simulink model "nms_sim_2D_cost"  (R2024b)
settings: Solver=ode15s  StartTime=0.0  StopTime=t_sim  MaxStep=dt_max  EnableMultiTasking=on
values from neighbouring files (symbols this model uses):
  a_BFSH = param_ctrl(35)*1    [setCtrlPar_optim_CPGreflex2001_2D.m]
  a_GAS = param_ctrl(37)*1    [setCtrlPar_optim_CPGreflex2001_2D.m]
  a_GLU = param_ctrl(31)*1    [setCtrlPar_optim_CPGreflex2001_2D.m]
  a_HAM = param_ctrl(33)*1    [setCtrlPar_optim_CPGreflex2001_2D.m]
  a_HFL = param_ctrl(32)*1    [setCtrlPar_optim_CPGreflex2001_2D.m]
  a_RF = param_ctrl(34)*1    [setCtrlPar_optim_CPGreflex2001_2D.m]
  a_SOL = param_ctrl(38)*1    [setCtrlPar_optim_CPGreflex2001_2D.m]
  a_TA = param_ctrl(39)*1    [setCtrlPar_optim_CPGreflex2001_2D.m]
  a_VAS = param_ctrl(36)*1    [setCtrlPar_optim_CPGreflex2001_2D.m]
  ai = param_ctrl(96)*2.0    [setCtrlPar_optim_CPGreflex2001_2D.m]
  b_BFSH = param_ctrl(52)*.51    [setCtrlPar_optim_CPGreflex2001_2D.m]
  b_BFSHGAS = param_ctrl(55)*.51    [setCtrlPar_optim_CPGreflex2001_2D.m]
  b_BFSHHAM = param_ctrl(54)*.51    [setCtrlPar_optim_CPGreflex2001_2D.m]
  b_BFSHVAS = param_ctrl(53)*.51    [setCtrlPar_optim_CPGreflex2001_2D.m]
  b_GAS = param_ctrl(59)*.51    [setCtrlPar_optim_CPGreflex2001_2D.m]
  b_GASBFSH = param_ctrl(60)*.51    [setCtrlPar_optim_CPGreflex2001_2D.m]
  b_GASSOL = param_ctrl(61)*.51    [setCtrlPar_optim_CPGreflex2001_2D.m]
  b_GLU = param_ctrl(40)*.51    [setCtrlPar_optim_CPGreflex2001_2D.m]
  b_GLUHAM = param_ctrl(42)*.51    [setCtrlPar_optim_CPGreflex2001_2D.m]
  b_GLUHFL = param_ctrl(41)*.51    [setCtrlPar_optim_CPGreflex2001_2D.m]
  b_HAM = param_ctrl(46)*.51    [setCtrlPar_optim_CPGreflex2001_2D.m]
  b_HAMBFSH = param_ctrl(48)*.51    [setCtrlPar_optim_CPGreflex2001_2D.m]
  b_HAMGLU = param_ctrl(47)*.51    [setCtrlPar_optim_CPGreflex2001_2D.m]
  b_HFL = param_ctrl(43)*.51    [setCtrlPar_optim_CPGreflex2001_2D.m]
  b_HFLGLU = param_ctrl(44)*.51    [setCtrlPar_optim_CPGreflex2001_2D.m]
  b_HFLRF = param_ctrl(45)*.51    [setCtrlPar_optim_CPGreflex2001_2D.m]
  b_RF = param_ctrl(49)*.51    [setCtrlPar_optim_CPGreflex2001_2D.m]
  b_RFHFL = param_ctrl(50)*.51    [setCtrlPar_optim_CPGreflex2001_2D.m]
  b_RFVAS = param_ctrl(51)*.51    [setCtrlPar_optim_CPGreflex2001_2D.m]
  b_SOL = param_ctrl(62)*.51    [setCtrlPar_optim_CPGreflex2001_2D.m]
  b_SOLGAS = param_ctrl(64)*.51    [setCtrlPar_optim_CPGreflex2001_2D.m]
  b_SOLTA = param_ctrl(63)*.51    [setCtrlPar_optim_CPGreflex2001_2D.m]
  b_TA = param_ctrl(65)*.51    [setCtrlPar_optim_CPGreflex2001_2D.m]
  b_TASOL = param_ctrl(66)*.51    [setCtrlPar_optim_CPGreflex2001_2D.m]
  b_VAS = param_ctrl(56)*.51    [setCtrlPar_optim_CPGreflex2001_2D.m]
  b_VASBFSH = param_ctrl(57)*.51    [setCtrlPar_optim_CPGreflex2001_2D.m]
  b_VASRF = param_ctrl(58)*.51    [setCtrlPar_optim_CPGreflex2001_2D.m]
  bias = param_ctrl(97)*2.5    [setCtrlPar_optim_CPGreflex2001_2D.m]
  c = 0.05    [nms_MS_2D_scaled.m]
  c_jointstop = 0.3 / (pi/180)    (= 17.1887338539)    [nms_MS_2D_scaled.m]
  D12_F = 0.16    *scaleL_JPhys    [nms_MechInit_2D_scaleSkel.m]
  D12_S = 0.2460	*sub_height    [nms_MechInit_2D_scaleSkel.m]
  D12_T = 0.2450  *sub_height    [nms_MechInit_2D_scaleSkel.m]
  D12y_F = 0.039  *sub_height    [nms_MechInit_2D_scaleSkel.m]
  D12z_HAT = 0.1    [nms_MS_2D_scaled.m]
  D13_F = 0.20    *scaleL_JPhys    [nms_MechInit_2D_scaleSkel.m]
  D1G_F = 0.14    *scaleL_JPhys    [nms_MechInit_2D_scaleSkel.m]
  D1G_HAT = 0.35  *scaleL_JPhys    [nms_MechInit_2D_scaleSkel.m]
  D1G_S = (0.3 - D12y_F/4)	*scaleL_JPhys    [nms_MechInit_2D_scaleSkel.m]
  D1G_T = (0.3 - D12y_F/4)	*scaleL_JPhys    [nms_MechInit_2D_scaleSkel.m]
  D1Gy_F = D12y_F*D1G_F/D12_F    (= 0.07)    [nms_MechInit_2D_scaleSkel.m]
  d_BFSH = param_ctrl(26)*1    [setCtrlPar_optim_CPGreflex2001_2D.m]
  d_GAS = param_ctrl(28)*1    [setCtrlPar_optim_CPGreflex2001_2D.m]
  d_GLU = param_ctrl(22)*1    [setCtrlPar_optim_CPGreflex2001_2D.m]
  d_HAM = param_ctrl(24)*1    [setCtrlPar_optim_CPGreflex2001_2D.m]
  d_HFL = param_ctrl(23)*1    [setCtrlPar_optim_CPGreflex2001_2D.m]
  d_RF = param_ctrl(25)*1    [setCtrlPar_optim_CPGreflex2001_2D.m]
  d_SOL = param_ctrl(29)*1    [setCtrlPar_optim_CPGreflex2001_2D.m]
  d_TA = param_ctrl(30)*1    [setCtrlPar_optim_CPGreflex2001_2D.m]
  d_VAS = param_ctrl(27)*1    [setCtrlPar_optim_CPGreflex2001_2D.m]
  DeltaThRef = 5e-3    (= 0.005)    [nms_MS_2D_scaled.m]
  dloptBFSH = 3.0    (= 3)    [setCtrlPar_optim_CPGreflex2001_2D.m]
  dloptGAS = 3.0    (= 3)    [setCtrlPar_optim_CPGreflex2001_2D.m]
  dloptGLU = 3.0    (= 3)    [setCtrlPar_optim_CPGreflex2001_2D.m]
  dloptHAM = 3.0    (= 3)    [setCtrlPar_optim_CPGreflex2001_2D.m]
  dloptHFL = 3.0    (= 3)    [setCtrlPar_optim_CPGreflex2001_2D.m]
  dloptRF = 3.0    (= 3)    [setCtrlPar_optim_CPGreflex2001_2D.m]
  dloptSOL = 3.0    (= 3)    [setCtrlPar_optim_CPGreflex2001_2D.m]
  dloptTA = 3.0    (= 3)    [setCtrlPar_optim_CPGreflex2001_2D.m]
  dloptVAS = 3.0    (= 3)    [setCtrlPar_optim_CPGreflex2001_2D.m]
  ec_BFSH = param_ctrl(80)*0.15    [setCtrlPar_optim_CPGreflex2001_2D.m]
  ec_GAS = param_ctrl(82)*0.15    [setCtrlPar_optim_CPGreflex2001_2D.m]
  ec_GLU = param_ctrl(76)*0.15    [setCtrlPar_optim_CPGreflex2001_2D.m]
  ec_HAM = param_ctrl(78)*0.15    [setCtrlPar_optim_CPGreflex2001_2D.m]
  ec_HFL = param_ctrl(77)*0.15    [setCtrlPar_optim_CPGreflex2001_2D.m]
  ec_RF = param_ctrl(79)*0.15    [setCtrlPar_optim_CPGreflex2001_2D.m]
  ec_TA = param_ctrl(84)*0.15    [setCtrlPar_optim_CPGreflex2001_2D.m]
  ec_VAS = param_ctrl(81)*0.15    [setCtrlPar_optim_CPGreflex2001_2D.m]
  eref = 0.04    [nms_MS_2D_scaled.m]
  eref_GAS = 0.1    [nms_MS_2D_scaled.m]
  eref_SOL = 0.1    [nms_MS_2D_scaled.m]
  es_BFSH = param_ctrl(89)*0.15    [setCtrlPar_optim_CPGreflex2001_2D.m]
  es_GAS = param_ctrl(91)*0.15    [setCtrlPar_optim_CPGreflex2001_2D.m]
  es_GLU = param_ctrl(85)*0.15    [setCtrlPar_optim_CPGreflex2001_2D.m]
  es_HAM = param_ctrl(87)*0.15    [setCtrlPar_optim_CPGreflex2001_2D.m]
  es_HFL = param_ctrl(86)*0.15    [setCtrlPar_optim_CPGreflex2001_2D.m]
  es_RF = param_ctrl(88)*0.15    [setCtrlPar_optim_CPGreflex2001_2D.m]
  es_TA = param_ctrl(93)*0.15    [setCtrlPar_optim_CPGreflex2001_2D.m]
  es_VAS = param_ctrl(90)*0.15    [setCtrlPar_optim_CPGreflex2001_2D.m]
  FmaxBFSH = 350    [nms_MS_2D_scaled.m]
  FmaxGAS = 2000    [nms_MS_2D_scaled.m]
  FmaxGLU = 4000    [nms_MS_2D_scaled.m]
  FmaxHAM = 2000    [nms_MS_2D_scaled.m]
  FmaxHFL = 2000    [nms_MS_2D_scaled.m]
  FmaxRF = 850    [nms_MS_2D_scaled.m]
  FmaxSOL = 4000    [nms_MS_2D_scaled.m]
  FmaxTA = 800    [nms_MS_2D_scaled.m]
  FmaxVAS = 5000    [nms_MS_2D_scaled.m]
  g = 9.81    [nms_MS_2D_scaled.m]
  gamma_4 = param_ctrl(11) * 1.7    [setCtrlPar_optim_CPGreflexsynergy2023_2D.m]
  h_BFSH = param_ctrl(71)*.1    [setCtrlPar_optim_CPGreflex2001_2D.m]
  h_GAS = param_ctrl(73)*.1    [setCtrlPar_optim_CPGreflex2001_2D.m]
  h_GLU = param_ctrl(67)*.1    [setCtrlPar_optim_CPGreflex2001_2D.m]
  h_HAM = param_ctrl(69)*.1    [setCtrlPar_optim_CPGreflex2001_2D.m]
  h_HFL = param_ctrl(68)*.1    [setCtrlPar_optim_CPGreflex2001_2D.m]
  h_RF = param_ctrl(70)*.1    [setCtrlPar_optim_CPGreflex2001_2D.m]
  h_SOL = param_ctrl(74)*.1    [setCtrlPar_optim_CPGreflex2001_2D.m]
  h_TA = param_ctrl(75)*.1    [setCtrlPar_optim_CPGreflex2001_2D.m]
  h_VAS = param_ctrl(72)*.1    [setCtrlPar_optim_CPGreflex2001_2D.m]
  HLCtrlPar = [theta_tgt l_clr alpha_tgt alpha_cd alpha_cv]    [setCtrlPar_optim_reflex2015_2D.m]
  In_F = 0.005    *scaleM*scaleL_JPhys^2    [nms_MechInit_2D_scaleSkel.m]
  In_HAT = 2.5    *scaleM*scaleL_JPhys^2    [nms_MechInit_2D_scaleSkel.m]
  In_S = 0.05     *scaleM*scaleL_JPhys^2    [nms_MechInit_2D_scaleSkel.m]
  In_T = 0.15     *scaleM*scaleL_JPhys^2    [nms_MechInit_2D_scaleSkel.m]
  init_exc = 0.01    [setInitPar_optim_2D.m]
  init_fm = 0.01    [setInitPar_optim_2D.m]
  init_lce = 1    [setInitPar_optim_2D.m]
  init_LCPG = param_ctrl(12) * 0.01    [setCtrlPar_optim_CPGreflexsynergy2023_2D.m]
  init_LStance = 1    [setInitPar_optim_2D.m]
  init_N1 = osc_signal1(phi_off_osc_ind)    [setCtrlPar_optim_CPGreflex2001_2D.m]
  ... (+441 more)
undefined symbols (not defined in the file or in its folder): cost_act_exponent, cost_v_tgt, flag_controller, Newton, nStep_obj, nStep_startKin, Raphson, sgn, SSW_kin, terrain_slope_angle, v_plateS1, X, Y, Z
libraries: nesl_utility x94, sm_lib x90, simulink x28, simulink_extras x12
(part 20 of 20)

== system nms_sim_2D_cost/Body Mechanics/RHeel Contact/2D Contact/Static Friction Model ==
  note: Stiction Limit Detector
  note: Static Friction Model
  note: Zero multiplication prevents
      | horizontal friction model from
      | oscillating between static and kinetic
      | friction when the vertical force is zero but
      | the ground level is not yet reached
      | in the upward motion
  note: (distance to
      | surface)
  note: Tangential Ground Reaction Force
  pos [m] : Inport
  vel [m/s m/s] : Inport  Port=2
  RefPtFP [m m] : Inport  Port=3
  posFP [m] : Inport  Port=4
  nVecFP [m m] : Inport  Port=5
  Enable : EnablePort  StatesWhenEnabling=reset  ZeroCross=off
  Abs : Abs  SaturateOnIntegerOverflow=off
  Check Vertical Friction : Product  RndMeth=Zero
  Constant : Constant
  Dpos_n : DotProduct  OutDataTypeStr=Inherit: Inherit via internal rule
  Dpos_nVec : Product  RndMeth=Zero
  Dpos_tVec : Sum  Inputs=|+-
  FixPt Relational Operator : RelationalOperator  Operator=>  OutDataTypeStr=boolean  ZeroCross=off  InputSameDT=off
  Gain : Gain  Gain=-1
  Gain1 : Gain  Gain=k_gn
  Gain2 : Gain  Gain=1/v_gn_max
  Gain3 : Gain  Gain=k_gt
  Gain5 : Gain  Gain=1/v_gt_max
  Memory : Memory
  Mux2 : Mux  Inputs=2
  Normal Ground Reaction Force : Fcn  Expr="u(1)  *  (1-u(2)) * (u(2)<1)"
  Positive : simulink/Logic and Bit Operations/Compare To Zero  relop=>  OutDataTypeStr=boolean
  Positive1 : simulink/Logic and Bit Operations/Compare To Zero  relop=>  OutDataTypeStr=boolean
  Product1 : Product  RndMeth=Zero
  Sign : Signum  ZeroCross=off
  Sum : Sum  Inputs=-+
  Sum1 : Sum  Inputs=|+-
  Sum2 : Sum  Inputs=|+-
  Vector Norm : Subsystem
  d_n : DotProduct  OutDataTypeStr=Inherit: Inherit via internal rule
  stiction limit force : Gain  Gain=mu_stick
  sum : Sum  Inputs=++|
  tVec1 : Product  Inputs=**  RndMeth=Zero
  tVec2 : Product  Inputs=**  RndMeth=Zero
  v_n : DotProduct  OutDataTypeStr=Inherit: Inherit via internal rule
  v_nVec : Product  RndMeth=Zero
  v_tVec : Sum  Inputs=-+|
  F_n Stick [N N] : Outport  OutputWhenDisabled=reset  InitialOutput=[0 0]  VectorParamsAs1DForOutWhenUnconnected=off
      settings: AttributesFormatString=initial = '%<InitialOutput>'\nwhen disabled = '%<OutputWhenDisabled>'
  F_t Stick [N N] : Outport  Port=2  OutputWhenDisabled=reset  InitialOutput=[0 0]  VectorParamsAs1DForOutWhenUnconnected=off
      settings: AttributesFormatString=when disabled: %<OutputWhenDisabled>\ninitial: %<InitialOutput>
  Sliding! : Outport  Port=3  OutputWhenDisabled=reset  InitialOutput=0  VectorParamsAs1DForOutWhenUnconnected=off
      settings: AttributesFormatString=when disabled: %<OutputWhenDisabled>\ninitial: %<InitialOutput>
  wires:
  Sum/1 -> Positive/1
  Memory/1 -> FixPt Relational Operator/2
  Positive/1 -> FixPt Relational Operator/1, Memory/1
  FixPt Relational Operator/1 -> Sliding!/1
  Abs/1 -> Sum/1
  stiction limit force/1 -> Abs/1
  Positive1/1 -> Check Vertical Friction/2
  Check Vertical Friction/1 -> Vector Norm/1(vec), F_t Stick [N N]/1
  Normal Ground Reaction Force/1 -> Product1/2, stiction limit force/1, Positive1/1
  Mux2/1 -> Normal Ground Reaction Force/1
  Gain1/1 -> Mux2/1
  Gain2/1 -> Mux2/2
  nVecFP [m m]/1 -> d_n/1, v_n/2, Dpos_n/1, Dpos_nVec/1, v_nVec/2, Product1/1
  d_n/1 -> Gain1/1
  vel [m/s m/s]/1 -> v_tVec/2, v_n/1
  v_n/1 -> v_nVec/1, Gain2/1
  v_nVec/1 -> v_tVec/1
  v_tVec/1 -> Gain5/1
  Product1/1 -> F_n Stick [N N]/1
  pos [m]/1 -> Sum2/1, Sum1/2
  posFP [m]/1 -> Sum2/2
  Sum2/1 -> Dpos_n/2, Dpos_tVec/1  "Dpos"
  Dpos_n/1 -> Dpos_nVec/2
  Dpos_nVec/1 -> Dpos_tVec/2
  Dpos_tVec/1 -> Gain3/1
  Gain3/1 -> Sign/1, tVec2/2
  Sign/1 -> tVec1/2
  tVec1/1 -> sum/2
  Constant/1 -> sum/1
  sum/1 -> tVec2/1
  tVec2/1 -> Gain/1
  Gain/1 -> Check Vertical Friction/1
  Vector Norm/1(norm) -> Sum/2
  RefPtFP [m m]/1 -> Sum1/1
  Sum1/1 -> d_n/2
  Gain5/1 -> tVec1/1

== system nms_sim_2D_cost/CPG-reflex-synergy controller/Central Pattern Generator/Left Central Pattern Generator/Pulse 0 ==
  phi out : Inport
  Constant : Constant  Value=u1
  Constant1 : Constant
  Cos : Trigonometry  Operator=cos
  Gain : Gain  Gain=pi/sigma1
  Gain1 : Gain  Gain=0.5
  Scope{,1..3} (4 alike) : Scope
  Sum : Sum  Inputs=|+-
  Sum1 : Sum  Inputs=|++
  Out1 : Outport
  wires:
  phi out/1 -> Sum/1
  Constant/1 -> Sum/2
  Sum/1 -> Scope/1, Gain/1
  Gain/1 -> Scope1/1, Cos/1
  Constant1/1 -> Sum1/2
  Cos/1 -> Scope2/1, Sum1/1
  Sum1/1 -> Scope3/1, Gain1/1
  Gain1/1 -> Out1/1

== system nms_sim_2D_cost/CPG-reflex-synergy controller/Central Pattern Generator/Left Central Pattern Generator/Pulse 1 ==
  phi out : Inport
  Constant : Constant  Value=u2
  Constant1 : Constant
  Cos : Trigonometry  Operator=cos
  Gain : Gain  Gain=pi/sigma2
  Gain1 : Gain  Gain=0.5
  Scope{,1..3} (4 alike) : Scope
  Sum : Sum  Inputs=|+-
  Sum1 : Sum  Inputs=|++
  Out1 : Outport
  wires:
  Gain1/1 -> Out1/1
  Sum1/1 -> Gain1/1, Scope3/1
  Cos/1 -> Sum1/1, Scope2/1
  Constant1/1 -> Sum1/2
  Gain/1 -> Cos/1, Scope1/1
  Sum/1 -> Gain/1, Scope/1
  Constant/1 -> Sum/2
  phi out/1 -> Sum/1

== system nms_sim_2D_cost/CPG-reflex-synergy controller/Central Pattern Generator/Left Central Pattern Generator/Pulse 2 ==
  phi out : Inport
  Constant : Constant  Value=u3
  Constant1 : Constant
  Cos : Trigonometry  Operator=cos
  Gain : Gain  Gain=pi/sigma3
  Gain1 : Gain  Gain=0.5
  Scope{,1..3} (4 alike) : Scope
  Sum : Sum  Inputs=|+-
  Sum1 : Sum  Inputs=|++
  Out1 : Outport
  wires:
  phi out/1 -> Sum/1
  Constant/1 -> Sum/2
  Sum/1 -> Scope/1, Gain/1
  Gain/1 -> Scope1/1, Cos/1
  Constant1/1 -> Sum1/2
  Cos/1 -> Scope2/1, Sum1/1
  Sum1/1 -> Scope3/1, Gain1/1
  Gain1/1 -> Out1/1

== system nms_sim_2D_cost/CPG-reflex-synergy controller/Central Pattern Generator/Left Central Pattern Generator/Pulse 3 ==
  phi out : Inport
  Constant : Constant  Value=u4
  Constant1 : Constant
  Cos : Trigonometry  Operator=cos
  Gain : Gain  Gain=pi/sigma4
  Gain1 : Gain  Gain=0.5
  Scope{,1..3} (4 alike) : Scope
  Sum : Sum  Inputs=|+-
  Sum1 : Sum  Inputs=|++
  Out1 : Outport
  wires:
  Gain1/1 -> Out1/1
  Sum1/1 -> Gain1/1, Scope3/1
  Cos/1 -> Sum1/1, Scope2/1
  Constant1/1 -> Sum1/2
  Gain/1 -> Cos/1, Scope1/1
  Sum/1 -> Gain/1, Scope/1
  Constant/1 -> Sum/2
  phi out/1 -> Sum/1

== system nms_sim_2D_cost/CPG-reflex-synergy controller/Central Pattern Generator/Left Central Pattern Generator/Pulse 4 ==
  phi out : Inport
  Constant : Constant  Value=u5
  Constant1 : Constant
  Cos : Trigonometry  Operator=cos
  Gain : Gain  Gain=pi/sigma5
  Gain1 : Gain  Gain=0.5
  Scope{,1..3} (4 alike) : Scope
  Sum : Sum  Inputs=|+-
  Sum1 : Sum  Inputs=|++
  Out1 : Outport
  wires:
  phi out/1 -> Sum/1
  Constant/1 -> Sum/2
  Sum/1 -> Scope/1, Gain/1
  Gain/1 -> Scope1/1, Cos/1
  Constant1/1 -> Sum1/2
  Cos/1 -> Scope2/1, Sum1/1
  Sum1/1 -> Scope3/1, Gain1/1
  Gain1/1 -> Out1/1

== system nms_sim_2D_cost/CPG-reflex-synergy controller/Central Pattern Generator/Right Central Pattern Generator/Pulse 0 ==
  phi out : Inport
  Constant : Constant  Value=u1
  Constant1 : Constant
  Cos : Trigonometry  Operator=cos
  Gain : Gain  Gain=pi/sigma1
  Gain1 : Gain  Gain=0.5
  Scope{,1..3} (4 alike) : Scope
  Sum : Sum  Inputs=|+-
  Sum1 : Sum  Inputs=|++
  Out1 : Outport
  wires:
  Gain1/1 -> Out1/1
  Sum1/1 -> Gain1/1, Scope3/1
  Cos/1 -> Sum1/1, Scope2/1
  Constant1/1 -> Sum1/2
  Gain/1 -> Cos/1, Scope1/1
  Sum/1 -> Gain/1, Scope/1
  Constant/1 -> Sum/2
  phi out/1 -> Sum/1

== system nms_sim_2D_cost/CPG-reflex-synergy controller/Central Pattern Generator/Right Central Pattern Generator/Pulse 1 ==
  phi out : Inport
  Constant : Constant  Value=u2
  Constant1 : Constant
  Cos : Trigonometry  Operator=cos
  Gain : Gain  Gain=pi/sigma2
  Gain1 : Gain  Gain=0.5
  Scope{,1..3} (4 alike) : Scope
  Sum : Sum  Inputs=|+-
  Sum1 : Sum  Inputs=|++
  Out1 : Outport
  wires:
  phi out/1 -> Sum/1
  Constant/1 -> Sum/2
  Sum/1 -> Scope/1, Gain/1
  Gain/1 -> Scope1/1, Cos/1
  Constant1/1 -> Sum1/2
  Cos/1 -> Scope2/1, Sum1/1
  Sum1/1 -> Scope3/1, Gain1/1
  Gain1/1 -> Out1/1

== system nms_sim_2D_cost/CPG-reflex-synergy controller/Central Pattern Generator/Right Central Pattern Generator/Pulse 2 ==
  phi out : Inport
  Constant : Constant  Value=u3
  Constant1 : Constant
  Cos : Trigonometry  Operator=cos
  Gain : Gain  Gain=pi/sigma3
  Gain1 : Gain  Gain=0.5
  Scope{,1..3} (4 alike) : Scope
  Sum : Sum  Inputs=|+-
  Sum1 : Sum  Inputs=|++
  Out1 : Outport
  wires:
  Gain1/1 -> Out1/1
  Sum1/1 -> Gain1/1, Scope3/1
  Cos/1 -> Sum1/1, Scope2/1
  Constant1/1 -> Sum1/2
  Gain/1 -> Cos/1, Scope1/1
  Sum/1 -> Gain/1, Scope/1
  Constant/1 -> Sum/2
  phi out/1 -> Sum/1

== system nms_sim_2D_cost/CPG-reflex-synergy controller/Central Pattern Generator/Right Central Pattern Generator/Pulse 3 ==
  phi out : Inport
  Constant : Constant  Value=u4
  Constant1 : Constant
  Cos : Trigonometry  Operator=cos
  Gain : Gain  Gain=pi/sigma4
  Gain1 : Gain  Gain=0.5
  Scope{,1..3} (4 alike) : Scope
  Sum : Sum  Inputs=|+-
  Sum1 : Sum  Inputs=|++
  Out1 : Outport
  wires:
  phi out/1 -> Sum/1
  Constant/1 -> Sum/2
  Sum/1 -> Scope/1, Gain/1
  Gain/1 -> Scope1/1, Cos/1
  Constant1/1 -> Sum1/2
  Cos/1 -> Scope2/1, Sum1/1
  Sum1/1 -> Scope3/1, Gain1/1
  Gain1/1 -> Out1/1

== system nms_sim_2D_cost/CPG-reflex-synergy controller/Central Pattern Generator/Right Central Pattern Generator/Pulse 4 ==
  phi out : Inport
  Constant : Constant  Value=u5
  Constant1 : Constant
  Cos : Trigonometry  Operator=cos
  Gain : Gain  Gain=pi/sigma5
  Gain1 : Gain  Gain=0.5
  Scope{,1..3} (4 alike) : Scope
  Sum : Sum  Inputs=|+-
  Sum1 : Sum  Inputs=|++
  Out1 : Outport
  wires:
  Gain1/1 -> Out1/1
  Sum1/1 -> Gain1/1, Scope3/1
  Cos/1 -> Sum1/1, Scope2/1
  Constant1/1 -> Sum1/2
  Gain/1 -> Cos/1, Scope1/1
  Sum/1 -> Gain/1, Scope/1
  Constant/1 -> Sum/2
  phi out/1 -> Sum/1

== system nms_sim_2D_cost/Reflex Controller/Lower Control Layer (Spinal Cord)/L Swing Phase/kneei_flexion from alpha ==
  note: Knee Phase i
  SBFSH : Inport
  Enable : EnablePort  StatesWhenEnabling=reset  ZeroCross=off
  SBFSH_Sw_ki : Outport  OutputWhenDisabled=reset  InitialOutput=0  VectorParamsAs1DForOutWhenUnconnected=off
  wires:
  SBFSH/1 -> SBFSH_Sw_ki/1

== system nms_sim_2D_cost/Reflex Controller/Lower Control Layer (Spinal Cord)/L Swing Phase/kneeii_damp and hold & kneeiii_leg stop & kneeiv_stance preparation ==
  note: Knee Phase i
  CtrlPar : Inport
  a_tgt : Inport  Port=2
  LceRF : Inport  Port=3
  LceHAM : Inport  Port=4
  VceHAM : Inport  Port=5
  VceVAS : Inport  Port=6
  VceBFSH : Inport  Port=7
  VceRF : Inport  Port=8
  LceHFL : Inport  Port=9
  LceGLU : Inport  Port=10
  LceVAS : Inport  Port=11
  Enable : EnablePort  StatesWhenEnabling=reset  ZeroCross=off
  Compare To Constant : simulink/Logic and Bit Operations/Compare To Constant  relop=<=  const=0  OutDataTypeStr=uint8  ZeroCross=off
  Constant1 : Constant  Value=0  OutDataTypeStr=boolean
  Constant2 : Constant  Value=0  OutDataTypeStr=boolean
  Constant3 : Constant  Value=0  OutDataTypeStr=boolean
  Constant4 : Constant
  Constant5 : Constant
  Demux1 : Demux  Outputs=5
  Divide1 : Product
  Divide2 : Product
  Logical Operator : Logic  Operator=NOT  AllPortsSameDT=off  OutDataTypeStr=boolean
  Logical Operator1 : Logic  AllPortsSameDT=off  OutDataTypeStr=boolean
  Relational Operator : RelationalOperator  Operator=<=  OutDataTypeStr=boolean  ZeroCross=off  InputSameDT=off
  Relational Operator1 : RelationalOperator  OutDataTypeStr=boolean  ZeroCross=off  InputSameDT=off
  S-R Flip-Flop : simulink_extras/Flip Flops/S-R Flip-Flop  initial_condition=0
  S-R Flip-Flop1 : simulink_extras/Flip Flops/S-R Flip-Flop  initial_condition=0
  S-R Flip-Flop2 : simulink_extras/Flip Flops/S-R Flip-Flop  initial_condition=0
  Sum1 : Sum  Inputs=+-|  InputSameDT=on  SaturateOnIntegerOverflow=on  OutDataTypeStr=Inherit: Same as first input
  Sum2 : Sum  Inputs=++|  InputSameDT=on  SaturateOnIntegerOverflow=on  OutDataTypeStr=Inherit: Same as first input
  Sum3 : Sum  Inputs=+-|  InputSameDT=on  SaturateOnIntegerOverflow=on  OutDataTypeStr=Inherit: Same as first input
  Sum4 : Sum  Inputs=+-|  InputSameDT=on  SaturateOnIntegerOverflow=on  OutDataTypeStr=Inherit: Same as first input
  Sum5 : Sum  Inputs=++|  InputSameDT=on  SaturateOnIntegerOverflow=on  OutDataTypeStr=Inherit: Same as first input
  Terminator : Terminator
  Terminator1 : Terminator
  Terminator2 : Terminator
  kneeii_damp and hold : Subsystem  TreatAsAtomicUnit=on
  kneeiii_leg stop : Subsystem  TreatAsAtomicUnit=on
  kneeiv_stance preparation : Subsystem  TreatAsAtomicUnit=on
  parSwKii : Selector  InputPortWidth=Sw_i  IndexOptions=Index vector (dialog)  Indices=parSwKii_i  OutputSizes=1
  parSwKiii : Selector  InputPortWidth=Sw_i  IndexOptions=Index vector (dialog)  Indices=parSwKiii_i  OutputSizes=1
  parSwKiv : Selector  InputPortWidth=Sw_i  IndexOptions=Index vector (dialog)  Indices=parSwKiv_i  OutputSizes=1
  parSwPhii : Selector  InputPortWidth=Sw_i  IndexOptions=Index vector (dialog)  Indices=parSwPhii_i  OutputSizes=1
  SRF_Sw_kii : Outport  OutputWhenDisabled=reset  InitialOutput=0  VectorParamsAs1DForOutWhenUnconnected=off
  SBFSH_Sw_kii : Outport  Port=2  OutputWhenDisabled=reset  InitialOutput=0  VectorParamsAs1DForOutWhenUnconnected=off
  SHAM_Sw_kiii : Outport  Port=3  OutputWhenDisabled=reset  InitialOutput=0  VectorParamsAs1DForOutWhenUnconnected=off
  SBFSH_Sw_kiii : Outport  Port=4  OutputWhenDisabled=reset  InitialOutput=0  VectorParamsAs1DForOutWhenUnconnected=off
  SGAS_Sw_kiii : Outport  Port=5  OutputWhenDisabled=reset  InitialOutput=0  VectorParamsAs1DForOutWhenUnconnected=off
  SHFL_Sw_kiv : Outport  Port=6  OutputWhenDisabled=reset  InitialOutput=0  VectorParamsAs1DForOutWhenUnconnected=off
  SGLU_Sw_kiv : Outport  Port=7  OutputWhenDisabled=reset  InitialOutput=0  VectorParamsAs1DForOutWhenUnconnected=off
  SVAS_Sw_kiv : Outport  Port=8  OutputWhenDisabled=reset  InitialOutput=0  VectorParamsAs1DForOutWhenUnconnected=off
  wires:
  Constant1/1 -> S-R Flip-Flop/2
  S-R Flip-Flop/2 -> Terminator/1
  Relational Operator/1 -> S-R Flip-Flop/1
  Constant2/1 -> S-R Flip-Flop1/2
  S-R Flip-Flop1/2 -> Terminator1/1
  Relational Operator1/1 -> S-R Flip-Flop1/1
  Constant3/1 -> S-R Flip-Flop2/2
  S-R Flip-Flop2/2 -> Terminator2/1
  Logical Operator1/1 -> S-R Flip-Flop2/1
  CtrlPar/1 -> parSwKii/1, parSwKiii/1, parSwKiv/1, parSwPhii/1
  S-R Flip-Flop/1 -> Logical Operator/1
  parSwKii/1 -> kneeii_damp and hold/1(CtrlPar)
  S-R Flip-Flop1/1 -> kneeiii_leg stop/Enable, Logical Operator1/1
  S-R Flip-Flop2/1 -> kneeiv_stance preparation/Enable
  parSwKiii/1 -> kneeiii_leg stop/1(CtrlPar)
  parSwKiv/1 -> kneeiv_stance preparation/1(CtrlPar)
  kneeii_damp and hold/1(SRF_Sw_kii) -> SRF_Sw_kii/1
  kneeii_damp and hold/2(SBFSH_Sw_kii) -> SBFSH_Sw_kii/1
  kneeiii_leg stop/1(SHAM_Sw_kiii) -> SHAM_Sw_kiii/1
  kneeiii_leg stop/2(SKFL_Sw_kiii) -> SBFSH_Sw_kiii/1
  kneeiii_leg stop/3(SGAS_Sw_kiii) -> SGAS_Sw_kiii/1
  kneeiv_stance preparation/1(SHFL_Sw_kiv) -> SHFL_Sw_kiv/1
  kneeiv_stance preparation/2(SGLU_Sw_kiv) -> SGLU_Sw_kiv/1
  kneeiv_stance preparation/3(SVAS_Sw_kiv) -> SVAS_Sw_kiv/1
  parSwPhii/1 -> Demux1/1
  Demux1/1 -> Sum3/2  "aRef_RF"
  Sum3/1 -> Divide1/1
  Constant4/1 -> Sum5/1
  Divide1/1 -> Sum5/2
  a_tgt/1 -> Sum2/1, Sum3/1, kneeii_damp and hold/2(a_tgt), kneeiii_leg stop/2(a_tgt), kneeiv_stance preparation/2(a_tgt)
  Demux1/2 -> Divide1/2  "a2lopt_RF"
  Sum5/1 -> Relational Operator/2  "lceOffRF"
  LceRF/1 -> Relational Operator/1, kneeii_damp and hold/6(LceRF)
  Logical Operator/1 -> kneeii_damp and hold/Enable
  Demux1/3 -> Sum2/2  "a_del"
  Sum2/1 -> Sum1/1  "a_thr"
  Demux1/4 -> Sum1/2  "aRef_HAM"
  Sum1/1 -> Divide2/1
  Demux1/5 -> Divide2/2  "a2lopt_HAM"
  Constant5/1 -> Sum4/1
  Divide2/1 -> Sum4/2
  Sum4/1 -> Relational Operator1/2  "lceOffHAM"
  LceHAM/1 -> kneeiii_leg stop/3(LceHAM), Relational Operator1/1  "LceHAM"
  Compare To Constant/1 -> Logical Operator1/2
  VceHAM/1 -> Compare To Constant/1
  VceBFSH/1 -> kneeii_damp and hold/4(VceBFSH)
  VceRF/1 -> kneeii_damp and hold/5(VceRF)
  LceHFL/1 -> kneeiv_stance preparation/3(LceHFL)
  LceGLU/1 -> kneeiv_stance preparation/4(lceGLU)
  LceVAS/1 -> kneeiv_stance preparation/5(lceVAS)
  VceVAS/1 -> kneeii_damp and hold/3(VceVAS)

== system nms_sim_2D_cost/Reflex Controller/Lower Control Layer (Spinal Cord)/R Swing Phase/kneei_flexion from alpha ==
  note: Knee Phase i
  SBFSH : Inport
  Enable : EnablePort  StatesWhenEnabling=reset  ZeroCross=off
  SBFSH_Sw_ki : Outport  OutputWhenDisabled=reset  InitialOutput=0  VectorParamsAs1DForOutWhenUnconnected=off
  wires:
  SBFSH/1 -> SBFSH_Sw_ki/1

== system nms_sim_2D_cost/Reflex Controller/Lower Control Layer (Spinal Cord)/R Swing Phase/kneeii_damp and hold & kneeiii_leg stop & kneeiv_stance preparation ==
  note: Knee Phase i
  CtrlPar : Inport
  a_tgt : Inport  Port=2
  LceRF : Inport  Port=3
  LceHAM : Inport  Port=4
  VceHAM : Inport  Port=5
  VceVAS : Inport  Port=6
  VceBFSH : Inport  Port=7
  VceRF : Inport  Port=8
  LceHFL : Inport  Port=9
  LceGLU : Inport  Port=10
  LceVAS : Inport  Port=11
  Enable : EnablePort  StatesWhenEnabling=reset  ZeroCross=off
  Compare To Constant : simulink/Logic and Bit Operations/Compare To Constant  relop=<=  const=0  OutDataTypeStr=uint8  ZeroCross=off
  Constant1 : Constant  Value=0  OutDataTypeStr=boolean
  Constant2 : Constant  Value=0  OutDataTypeStr=boolean
  Constant3 : Constant  Value=0  OutDataTypeStr=boolean
  Constant4 : Constant
  Constant5 : Constant
  Demux1 : Demux  Outputs=5
  Divide1 : Product
  Divide2 : Product
  Logical Operator : Logic  Operator=NOT  AllPortsSameDT=off  OutDataTypeStr=boolean
  Logical Operator1 : Logic  AllPortsSameDT=off  OutDataTypeStr=boolean
  Relational Operator : RelationalOperator  Operator=<=  OutDataTypeStr=boolean  ZeroCross=off  InputSameDT=off
  Relational Operator1 : RelationalOperator  OutDataTypeStr=boolean  ZeroCross=off  InputSameDT=off
  S-R Flip-Flop : simulink_extras/Flip Flops/S-R Flip-Flop  initial_condition=0
  S-R Flip-Flop1 : simulink_extras/Flip Flops/S-R Flip-Flop  initial_condition=0
  S-R Flip-Flop2 : simulink_extras/Flip Flops/S-R Flip-Flop  initial_condition=0
  Sum1 : Sum  Inputs=+-|  InputSameDT=on  SaturateOnIntegerOverflow=on  OutDataTypeStr=Inherit: Same as first input
  Sum2 : Sum  Inputs=++|  InputSameDT=on  SaturateOnIntegerOverflow=on  OutDataTypeStr=Inherit: Same as first input
  Sum3 : Sum  Inputs=+-|  InputSameDT=on  SaturateOnIntegerOverflow=on  OutDataTypeStr=Inherit: Same as first input
  Sum4 : Sum  Inputs=+-|  InputSameDT=on  SaturateOnIntegerOverflow=on  OutDataTypeStr=Inherit: Same as first input
  Sum5 : Sum  Inputs=++|  InputSameDT=on  SaturateOnIntegerOverflow=on  OutDataTypeStr=Inherit: Same as first input
  Terminator : Terminator
  Terminator1 : Terminator
  Terminator2 : Terminator
  kneeii_damp and hold : Subsystem  TreatAsAtomicUnit=on
  kneeiii_leg stop : Subsystem  TreatAsAtomicUnit=on
  kneeiv_stance preparation : Subsystem  TreatAsAtomicUnit=on
  parSwKii : Selector  InputPortWidth=Sw_i  IndexOptions=Index vector (dialog)  Indices=parSwKii_i  OutputSizes=1
  parSwKiii : Selector  InputPortWidth=Sw_i  IndexOptions=Index vector (dialog)  Indices=parSwKiii_i  OutputSizes=1
  parSwKiv : Selector  InputPortWidth=Sw_i  IndexOptions=Index vector (dialog)  Indices=parSwKiv_i  OutputSizes=1
  parSwPhii : Selector  InputPortWidth=Sw_i  IndexOptions=Index vector (dialog)  Indices=parSwPhii_i  OutputSizes=1
  SRF_Sw_kii : Outport  OutputWhenDisabled=reset  InitialOutput=0  VectorParamsAs1DForOutWhenUnconnected=off
  SBFSH_Sw_kii : Outport  Port=2  OutputWhenDisabled=reset  InitialOutput=0  VectorParamsAs1DForOutWhenUnconnected=off
  SHAM_Sw_kiii : Outport  Port=3  OutputWhenDisabled=reset  InitialOutput=0  VectorParamsAs1DForOutWhenUnconnected=off
  SBFSH_Sw_kiii : Outport  Port=4  OutputWhenDisabled=reset  InitialOutput=0  VectorParamsAs1DForOutWhenUnconnected=off
  SGAS_Sw_kiii : Outport  Port=5  OutputWhenDisabled=reset  InitialOutput=0  VectorParamsAs1DForOutWhenUnconnected=off
  SHFL_Sw_kiv : Outport  Port=6  OutputWhenDisabled=reset  InitialOutput=0  VectorParamsAs1DForOutWhenUnconnected=off
  SGLU_Sw_kiv : Outport  Port=7  OutputWhenDisabled=reset  InitialOutput=0  VectorParamsAs1DForOutWhenUnconnected=off
  SVAS_Sw_kiv : Outport  Port=8  OutputWhenDisabled=reset  InitialOutput=0  VectorParamsAs1DForOutWhenUnconnected=off
  wires:
  Constant1/1 -> S-R Flip-Flop/2
  S-R Flip-Flop/2 -> Terminator/1
  Relational Operator/1 -> S-R Flip-Flop/1
  Constant2/1 -> S-R Flip-Flop1/2
  S-R Flip-Flop1/2 -> Terminator1/1
  Relational Operator1/1 -> S-R Flip-Flop1/1
  Constant3/1 -> S-R Flip-Flop2/2
  S-R Flip-Flop2/2 -> Terminator2/1
  Logical Operator1/1 -> S-R Flip-Flop2/1
  CtrlPar/1 -> parSwKii/1, parSwKiii/1, parSwKiv/1, parSwPhii/1
  S-R Flip-Flop/1 -> Logical Operator/1
  parSwKii/1 -> kneeii_damp and hold/1(CtrlPar)
  S-R Flip-Flop1/1 -> kneeiii_leg stop/Enable, Logical Operator1/1
  S-R Flip-Flop2/1 -> kneeiv_stance preparation/Enable
  parSwKiii/1 -> kneeiii_leg stop/1(CtrlPar)
  parSwKiv/1 -> kneeiv_stance preparation/1(CtrlPar)
  kneeii_damp and hold/1(SRF_Sw_kii) -> SRF_Sw_kii/1
  kneeii_damp and hold/2(SBFSH_Sw_kii) -> SBFSH_Sw_kii/1
  kneeiii_leg stop/1(SHAM_Sw_kiii) -> SHAM_Sw_kiii/1
  kneeiii_leg stop/2(SKFL_Sw_kiii) -> SBFSH_Sw_kiii/1
  kneeiii_leg stop/3(SGAS_Sw_kiii) -> SGAS_Sw_kiii/1
  kneeiv_stance preparation/1(SHFL_Sw_kiv) -> SHFL_Sw_kiv/1
  kneeiv_stance preparation/2(SGLU_Sw_kiv) -> SGLU_Sw_kiv/1
  kneeiv_stance preparation/3(SVAS_Sw_kiv) -> SVAS_Sw_kiv/1
  parSwPhii/1 -> Demux1/1
  Demux1/1 -> Sum3/2  "aRef_RF"
  Sum3/1 -> Divide1/1
  Constant4/1 -> Sum5/1
  Divide1/1 -> Sum5/2
  a_tgt/1 -> Sum2/1, Sum3/1, kneeii_damp and hold/2(a_tgt), kneeiii_leg stop/2(a_tgt), kneeiv_stance preparation/2(a_tgt)
  Demux1/2 -> Divide1/2  "a2lopt_RF"
  Sum5/1 -> Relational Operator/2  "lceOffRF"
  LceRF/1 -> Relational Operator/1, kneeii_damp and hold/6(LceRF)
  Logical Operator/1 -> kneeii_damp and hold/Enable
  Demux1/3 -> Sum2/2  "a_del"
  Sum2/1 -> Sum1/1  "a_thr"
  Demux1/4 -> Sum1/2  "aRef_HAM"
  Sum1/1 -> Divide2/1
  Demux1/5 -> Divide2/2  "a2lopt_HAM"
  Constant5/1 -> Sum4/1
  Divide2/1 -> Sum4/2
  Sum4/1 -> Relational Operator1/2  "lceOffHAM"
  LceHAM/1 -> kneeiii_leg stop/3(LceHAM), Relational Operator1/1  "LceHAM"
  Compare To Constant/1 -> Logical Operator1/2
  VceHAM/1 -> Compare To Constant/1
  VceBFSH/1 -> kneeii_damp and hold/4(VceBFSH)
  VceRF/1 -> kneeii_damp and hold/5(VceRF)
  LceHFL/1 -> kneeiv_stance preparation/3(LceHFL)
  LceGLU/1 -> kneeiv_stance preparation/4(lceGLU)
  LceVAS/1 -> kneeiv_stance preparation/5(lceVAS)
  VceVAS/1 -> kneeii_damp and hold/3(VceVAS)

== system nms_sim_2D_cost/Body Mechanics/LBall Contact/2D Contact/Kinetic Friction Model/Vector Norm ==
  vec : Inport
  Sqrt : Sqrt  OutputSignalType=real  AlgorithmType=Newton-Raphson
  Squares : Math  Operator=square  SignedPower=on  OutputSignalType=real
  Sum of Elements : Sum  Inputs=+
  norm : Outport  VectorParamsAs1DForOutWhenUnconnected=off
  wires:
  vec/1 -> Squares/1
  Sqrt/1 -> norm/1
  Sum of Elements/1 -> Sqrt/1
  Squares/1 -> Sum of Elements/1

== system nms_sim_2D_cost/Body Mechanics/LBall Contact/2D Contact/Static Friction Model/Vector Norm ==
  vec : Inport
  Sqrt : Sqrt  OutputSignalType=real  AlgorithmType=Newton-Raphson
  Squares : Math  Operator=square  SignedPower=on  OutputSignalType=real
  Sum of Elements : Sum  Inputs=+
  norm : Outport  VectorParamsAs1DForOutWhenUnconnected=off
  wires:
  vec/1 -> Squares/1
  Sqrt/1 -> norm/1
  Sum of Elements/1 -> Sqrt/1
  Squares/1 -> Sum of Elements/1

== system nms_sim_2D_cost/Body Mechanics/LHeel Contact/2D Contact/Kinetic Friction Model/Vector Norm ==
  vec : Inport
  Sqrt : Sqrt  OutputSignalType=real  AlgorithmType=Newton-Raphson
  Squares : Math  Operator=square  SignedPower=on  OutputSignalType=real
  Sum of Elements : Sum  Inputs=+
  norm : Outport  VectorParamsAs1DForOutWhenUnconnected=off
  wires:
  vec/1 -> Squares/1
  Sqrt/1 -> norm/1
  Sum of Elements/1 -> Sqrt/1
  Squares/1 -> Sum of Elements/1

== system nms_sim_2D_cost/Body Mechanics/LHeel Contact/2D Contact/Static Friction Model/Vector Norm ==
  vec : Inport
  Sqrt : Sqrt  OutputSignalType=real  AlgorithmType=Newton-Raphson
  Squares : Math  Operator=square  SignedPower=on  OutputSignalType=real
  Sum of Elements : Sum  Inputs=+
  norm : Outport  VectorParamsAs1DForOutWhenUnconnected=off
  wires:
  vec/1 -> Squares/1
  Sqrt/1 -> norm/1
  Sum of Elements/1 -> Sqrt/1
  Squares/1 -> Sum of Elements/1

== system nms_sim_2D_cost/Body Mechanics/RBall Contact/2D Contact/Kinetic Friction Model/Vector Norm ==
  vec : Inport
  Sqrt : Sqrt  OutputSignalType=real  AlgorithmType=Newton-Raphson
  Squares : Math  Operator=square  SignedPower=on  OutputSignalType=real
  Sum of Elements : Sum  Inputs=+
  norm : Outport  VectorParamsAs1DForOutWhenUnconnected=off
  wires:
  vec/1 -> Squares/1
  Sqrt/1 -> norm/1
  Sum of Elements/1 -> Sqrt/1
  Squares/1 -> Sum of Elements/1

== system nms_sim_2D_cost/Body Mechanics/RBall Contact/2D Contact/Static Friction Model/Vector Norm ==
  vec : Inport
  Sqrt : Sqrt  OutputSignalType=real  AlgorithmType=Newton-Raphson
  Squares : Math  Operator=square  SignedPower=on  OutputSignalType=real
  Sum of Elements : Sum  Inputs=+
  norm : Outport  VectorParamsAs1DForOutWhenUnconnected=off
  wires:
  vec/1 -> Squares/1
  Sqrt/1 -> norm/1
  Sum of Elements/1 -> Sqrt/1
  Squares/1 -> Sum of Elements/1

== system nms_sim_2D_cost/Body Mechanics/RHeel Contact/2D Contact/Kinetic Friction Model/Vector Norm ==
  vec : Inport
  Sqrt : Sqrt  OutputSignalType=real  AlgorithmType=Newton-Raphson
  Squares : Math  Operator=square  SignedPower=on  OutputSignalType=real
  Sum of Elements : Sum  Inputs=+
  norm : Outport  VectorParamsAs1DForOutWhenUnconnected=off
  wires:
  vec/1 -> Squares/1
  Sqrt/1 -> norm/1
  Sum of Elements/1 -> Sqrt/1
  Squares/1 -> Sum of Elements/1

== system nms_sim_2D_cost/Body Mechanics/RHeel Contact/2D Contact/Static Friction Model/Vector Norm ==
  vec : Inport
  Sqrt : Sqrt  OutputSignalType=real  AlgorithmType=Newton-Raphson
  Squares : Math  Operator=square  SignedPower=on  OutputSignalType=real
  Sum of Elements : Sum  Inputs=+
  norm : Outport  VectorParamsAs1DForOutWhenUnconnected=off
  wires:
  vec/1 -> Squares/1
  Sqrt/1 -> norm/1
  Sum of Elements/1 -> Sqrt/1
  Squares/1 -> Sum of Elements/1

== system nms_sim_2D_cost/Reflex Controller/Lower Control Layer (Spinal Cord)/L Swing Phase/kneeii_damp and hold & kneeiii_leg stop & kneeiv_stance preparation/kneeii_damp and hold ==
  note: Knee Phase i
  CtrlPar : Inport
  a_tgt : Inport  Port=2
  VceVAS : Inport  Port=3
  VceBFSH : Inport  Port=4
  VceRF : Inport  Port=5
  LceRF : Inport  Port=6
  Enable : EnablePort  StatesWhenEnabling=reset  ZeroCross=off
  Constant5 : Constant
  Demux2 : Demux  Outputs=5
  Divide1 : Product
  Divide2 : Product  Inputs=3
  Divide3 : Product  Inputs=*/
  Divide4 : Product  Inputs=*/
  Divide5 : Product
  Divide6 : Product
  Divide7 : Product  Inputs=*/
  Sum1 : Sum  Inputs=|-+  InputSameDT=on  SaturateOnIntegerOverflow=on  OutDataTypeStr=Inherit: Same as first input
  Sum10 : Sum  Inputs=|++  InputSameDT=on  SaturateOnIntegerOverflow=on  OutDataTypeStr=Inherit: Same as first input
  Sum2 : Sum  Inputs=|+-  InputSameDT=on  SaturateOnIntegerOverflow=on  OutDataTypeStr=Inherit: Same as first input
  Sum7 : Sum  Inputs=++|  InputSameDT=on  SaturateOnIntegerOverflow=on  OutDataTypeStr=Inherit: Same as first input
  positive half{,1..3} (4 alike) : Saturate  UpperLimit=inf  LowerLimit=0  ZeroCross=off
  SRF_Sw_kii : Outport  OutputWhenDisabled=reset  InitialOutput=0  VectorParamsAs1DForOutWhenUnconnected=off
  SBFSH_Sw_kii : Outport  Port=2  OutputWhenDisabled=reset  InitialOutput=0  VectorParamsAs1DForOutWhenUnconnected=off
  wires:
  CtrlPar/1 -> Demux2/1
  Demux2/1 -> Divide5/2  "VGainVAS_RF"
  VceBFSH/1 -> positive half/1, Divide3/1
  Divide5/1 -> SRF_Sw_kii/1
  positive half3/1 -> Divide5/1
  positive half/1 -> Divide1/1
  Demux2/2 -> Divide1/2  "VGainBFSH"
  Divide1/1 -> Divide2/1
  positive half1/1 -> Divide2/2
  Demux2/3 -> Divide3/2  "phi2lopt_BFSH"
  VceRF/1 -> Divide4/1
  Demux2/4 -> Divide4/2, Divide6/1, Divide7/2  "a2lopt_RF"
  Divide4/1 -> Sum7/2
  Divide3/1 -> Sum7/1
  Sum7/1 -> positive half1/1
  positive half2/1 -> Divide2/3
  a_tgt/1 -> Sum1/2
  Demux2/5 -> Sum1/1  "aRef_RF"
  Sum1/1 -> Divide6/2
  Divide6/1 -> Sum10/1
  Constant5/1 -> Sum10/2
  Sum10/1 -> Sum2/1  "lceOffRF"
  LceRF/1 -> Sum2/2
  Sum2/1 -> Divide7/1
  Divide7/1 -> positive half2/1
  Divide2/1 -> SBFSH_Sw_kii/1
  VceVAS/1 -> positive half3/1

== system nms_sim_2D_cost/Reflex Controller/Lower Control Layer (Spinal Cord)/L Swing Phase/kneeii_damp and hold & kneeiii_leg stop & kneeiv_stance preparation/kneeiii_leg stop ==
  note: Knee Phase iii
  CtrlPar : Inport
  a_tgt : Inport  Port=2
  LceHAM : Inport  Port=3
  Enable : EnablePort  StatesWhenEnabling=reset  ZeroCross=off
  Constant5 : Constant
  Demux1 : Demux  Outputs=7
  Divide{1..2,5,22} (4 alike) : Product
  Sum1 : Sum  Inputs=-+|  InputSameDT=on  SaturateOnIntegerOverflow=on  OutDataTypeStr=Inherit: Same as first input
  Sum10 : Sum  Inputs=+-|  InputSameDT=on  SaturateOnIntegerOverflow=on  OutDataTypeStr=Inherit: Same as first input
  Sum2 : Sum  Inputs=++|  InputSameDT=on  SaturateOnIntegerOverflow=on  OutDataTypeStr=Inherit: Same as first input
  Sum3 : Sum  Inputs=+-|  InputSameDT=on  SaturateOnIntegerOverflow=on  OutDataTypeStr=Inherit: Same as first input
  Sum4 : Sum  Inputs=+-|  InputSameDT=on  SaturateOnIntegerOverflow=on  OutDataTypeStr=Inherit: Same as first input
  positive half1 : Saturate  UpperLimit=inf  LowerLimit=0  ZeroCross=off
  positive half2 : Saturate  UpperLimit=inf  LowerLimit=0  ZeroCross=off
  SHAM_Sw_kiii : Outport  OutputWhenDisabled=reset  InitialOutput=0  VectorParamsAs1DForOutWhenUnconnected=off
  SKFL_Sw_kiii : Outport  Port=2  OutputWhenDisabled=reset  InitialOutput=0  VectorParamsAs1DForOutWhenUnconnected=off
  SGAS_Sw_kiii : Outport  Port=3  OutputWhenDisabled=reset  InitialOutput=0  VectorParamsAs1DForOutWhenUnconnected=off
  wires:
  CtrlPar/1 -> Demux1/1
  Sum1/1 -> positive half2/1  "del_LceMAN"
  LceHAM/1 -> Sum1/2  "LceHAM"
  positive half2/1 -> Divide5/1  "del_lce"
  Constant5/1 -> Sum10/1
  Divide22/1 -> Sum10/2
  a_tgt/1 -> Sum2/1
  Demux1/1 -> Sum2/2  "a_del"
  Sum2/1 -> Sum3/1  "a_thr"
  Demux1/2 -> Sum3/2  "aRef_HAM"
  Sum3/1 -> Divide22/1
  Demux1/3 -> Divide22/2  "a2lopt_HAM"
  Sum10/1 -> Sum1/1  "lceOffHAM"
  Demux1/4 -> Divide5/2  "LGainHAM"
  Divide5/1 -> Sum4/1, SHAM_Sw_kiii/1  "S_HAM"
  Sum4/1 -> positive half1/1
  Demux1/5 -> Sum4/2  "SHAM_thr"
  positive half1/1 -> Divide1/1, Divide2/1
  Demux1/6 -> Divide1/2  "SGainHAM_KFL"
  Divide1/1 -> SKFL_Sw_kiii/1
  Divide2/1 -> SGAS_Sw_kiii/1
  Demux1/7 -> Divide2/2  "SGainHAM_GAS"

== system nms_sim_2D_cost/Reflex Controller/Lower Control Layer (Spinal Cord)/L Swing Phase/kneeii_damp and hold & kneeiii_leg stop & kneeiv_stance preparation/kneeiv_stance preparation ==
  note: Knee Phase iii
  CtrlPar : Inport
  a_tgt : Inport  Port=2
  LceHFL : Inport  Port=3
  lceGLU : Inport  Port=4
  lceVAS : Inport  Port=5
  Enable : EnablePort  StatesWhenEnabling=reset  ZeroCross=off
  Constant1 : Constant
  Constant2 : Constant
  Constant5 : Constant  Value=pi/2
  Demux2 : Demux  Outputs=8
  Divide{1..3,5..6} (5 alike) : Product
  Sum1 : Sum  Inputs=-+|  InputSameDT=on  SaturateOnIntegerOverflow=on  OutDataTypeStr=Inherit: Same as first input
  Sum2 : Sum  Inputs=++|  InputSameDT=on  SaturateOnIntegerOverflow=on  OutDataTypeStr=Inherit: Same as first input
  Sum3 : Sum  Inputs=+-|  InputSameDT=on  SaturateOnIntegerOverflow=on  OutDataTypeStr=Inherit: Same as first input
  Sum4 : Sum  Inputs=+-|  InputSameDT=on  SaturateOnIntegerOverflow=on  OutDataTypeStr=Inherit: Same as first input
  Sum5 : Sum  Inputs=++|  InputSameDT=on  SaturateOnIntegerOverflow=on  OutDataTypeStr=Inherit: Same as first input
  Sum6 : Sum  Inputs=-+|  InputSameDT=on  SaturateOnIntegerOverflow=on  OutDataTypeStr=Inherit: Same as first input
  Sum7 : Sum  Inputs=+-|  InputSameDT=on  SaturateOnIntegerOverflow=on  OutDataTypeStr=Inherit: Same as first input
  Sum9 : Sum  Inputs=-+|  InputSameDT=on  SaturateOnIntegerOverflow=on  OutDataTypeStr=Inherit: Same as first input
  positive half1 : Saturate  UpperLimit=inf  LowerLimit=0  ZeroCross=off
  positive half2 : Saturate  UpperLimit=inf  LowerLimit=0  ZeroCross=off
  positive half3 : Saturate  UpperLimit=inf  LowerLimit=0  ZeroCross=off
  SHFL_Sw_kiv : Outport  OutputWhenDisabled=reset  InitialOutput=0  VectorParamsAs1DForOutWhenUnconnected=off
  SGLU_Sw_kiv : Outport  Port=2  OutputWhenDisabled=reset  InitialOutput=0  VectorParamsAs1DForOutWhenUnconnected=off
  SVAS_Sw_kiv : Outport  Port=3  OutputWhenDisabled=reset  InitialOutput=0  VectorParamsAs1DForOutWhenUnconnected=off
  wires:
  CtrlPar/1 -> Demux2/1
  Sum1/1 -> positive half2/1
  LceHFL/1 -> Sum1/2
  positive half2/1 -> Divide5/1
  a_tgt/1 -> Sum2/2
  Constant5/1 -> Sum2/1
  Demux2/1 -> Sum3/2  "phiRef_HFL"
  Sum2/1 -> Sum3/1, Sum4/1
  Sum3/1 -> Divide1/1
  Demux2/2 -> Divide1/2  "phi2lopt_HFL"
  Demux2/5 -> Divide2/2  "phi2lopt_GLU"
  Demux2/4 -> Sum4/2  "phiRef_GLU"
  Sum4/1 -> Divide2/1
  Demux2/3 -> Divide5/2  "LGainHFL"
  Divide5/1 -> SHFL_Sw_kiv/1
  Constant1/1 -> Sum5/1
  Divide1/1 -> Sum5/2
  Sum5/1 -> Sum1/1  "lceOffHFL"
  Sum6/1 -> positive half1/1  "del_lce"
  lceGLU/1 -> Sum6/2  "lceGLU"
  positive half1/1 -> Divide3/1
  Demux2/6 -> Divide3/2  "LGainGLU"
  Divide3/1 -> SGLU_Sw_kiv/1
  Constant2/1 -> Sum7/1
  Divide2/1 -> Sum7/2
  Sum7/1 -> Sum6/1  "lceOffGLU"
  Sum9/1 -> positive half3/1
  lceVAS/1 -> Sum9/2
  positive half3/1 -> Divide6/1
  Divide6/1 -> SVAS_Sw_kiv/1
  Demux2/7 -> Sum9/1  "loffVAS"
  Demux2/8 -> Divide6/2  "LGainVAS"

== system nms_sim_2D_cost/Reflex Controller/Lower Control Layer (Spinal Cord)/R Swing Phase/kneeii_damp and hold & kneeiii_leg stop & kneeiv_stance preparation/kneeii_damp and hold ==
  note: Knee Phase i
  CtrlPar : Inport
  a_tgt : Inport  Port=2
  VceVAS : Inport  Port=3
  VceBFSH : Inport  Port=4
  VceRF : Inport  Port=5
  LceRF : Inport  Port=6
  Enable : EnablePort  StatesWhenEnabling=reset  ZeroCross=off
  Constant5 : Constant
  Demux2 : Demux  Outputs=5
  Divide1 : Product
  Divide2 : Product  Inputs=3
  Divide3 : Product  Inputs=*/
  Divide4 : Product  Inputs=*/
  Divide5 : Product
  Divide6 : Product
  Divide7 : Product  Inputs=*/
  Sum1 : Sum  Inputs=|-+  InputSameDT=on  SaturateOnIntegerOverflow=on  OutDataTypeStr=Inherit: Same as first input
  Sum10 : Sum  Inputs=|++  InputSameDT=on  SaturateOnIntegerOverflow=on  OutDataTypeStr=Inherit: Same as first input
  Sum2 : Sum  Inputs=|+-  InputSameDT=on  SaturateOnIntegerOverflow=on  OutDataTypeStr=Inherit: Same as first input
  Sum7 : Sum  Inputs=++|  InputSameDT=on  SaturateOnIntegerOverflow=on  OutDataTypeStr=Inherit: Same as first input
  positive half{,1..3} (4 alike) : Saturate  UpperLimit=inf  LowerLimit=0  ZeroCross=off
  SRF_Sw_kii : Outport  OutputWhenDisabled=reset  InitialOutput=0  VectorParamsAs1DForOutWhenUnconnected=off
  SBFSH_Sw_kii : Outport  Port=2  OutputWhenDisabled=reset  InitialOutput=0  VectorParamsAs1DForOutWhenUnconnected=off
  wires:
  CtrlPar/1 -> Demux2/1
  Demux2/1 -> Divide5/2  "VGainVAS_RF"
  VceBFSH/1 -> positive half/1, Divide3/1
  Divide5/1 -> SRF_Sw_kii/1
  positive half3/1 -> Divide5/1
  positive half/1 -> Divide1/1
  Demux2/2 -> Divide1/2  "VGainBFSH"
  Divide1/1 -> Divide2/1
  positive half1/1 -> Divide2/2
  Demux2/3 -> Divide3/2  "phi2lopt_BFSH"
  VceRF/1 -> Divide4/1
  Demux2/4 -> Divide4/2, Divide6/1, Divide7/2  "a2lopt_RF"
  Divide4/1 -> Sum7/2
  Divide3/1 -> Sum7/1
  Sum7/1 -> positive half1/1
  positive half2/1 -> Divide2/3
  a_tgt/1 -> Sum1/2
  Demux2/5 -> Sum1/1  "aRef_RF"
  Sum1/1 -> Divide6/2
  Divide6/1 -> Sum10/1
  Constant5/1 -> Sum10/2
  Sum10/1 -> Sum2/1  "lceOffRF"
  LceRF/1 -> Sum2/2
  Sum2/1 -> Divide7/1
  Divide7/1 -> positive half2/1
  Divide2/1 -> SBFSH_Sw_kii/1
  VceVAS/1 -> positive half3/1

== system nms_sim_2D_cost/Reflex Controller/Lower Control Layer (Spinal Cord)/R Swing Phase/kneeii_damp and hold & kneeiii_leg stop & kneeiv_stance preparation/kneeiii_leg stop ==
  note: Knee Phase iii
  CtrlPar : Inport
  a_tgt : Inport  Port=2
  LceHAM : Inport  Port=3
  Enable : EnablePort  StatesWhenEnabling=reset  ZeroCross=off
  Constant5 : Constant
  Demux1 : Demux  Outputs=7
  Divide{1..2,5,22} (4 alike) : Product
  Sum1 : Sum  Inputs=-+|  InputSameDT=on  SaturateOnIntegerOverflow=on  OutDataTypeStr=Inherit: Same as first input
  Sum10 : Sum  Inputs=+-|  InputSameDT=on  SaturateOnIntegerOverflow=on  OutDataTypeStr=Inherit: Same as first input
  Sum2 : Sum  Inputs=++|  InputSameDT=on  SaturateOnIntegerOverflow=on  OutDataTypeStr=Inherit: Same as first input
  Sum3 : Sum  Inputs=+-|  InputSameDT=on  SaturateOnIntegerOverflow=on  OutDataTypeStr=Inherit: Same as first input
  Sum4 : Sum  Inputs=+-|  InputSameDT=on  SaturateOnIntegerOverflow=on  OutDataTypeStr=Inherit: Same as first input
  positive half1 : Saturate  UpperLimit=inf  LowerLimit=0  ZeroCross=off
  positive half2 : Saturate  UpperLimit=inf  LowerLimit=0  ZeroCross=off
  SHAM_Sw_kiii : Outport  OutputWhenDisabled=reset  InitialOutput=0  VectorParamsAs1DForOutWhenUnconnected=off
  SKFL_Sw_kiii : Outport  Port=2  OutputWhenDisabled=reset  InitialOutput=0  VectorParamsAs1DForOutWhenUnconnected=off
  SGAS_Sw_kiii : Outport  Port=3  OutputWhenDisabled=reset  InitialOutput=0  VectorParamsAs1DForOutWhenUnconnected=off
  wires:
  CtrlPar/1 -> Demux1/1
  Sum1/1 -> positive half2/1  "del_LceMAN"
  LceHAM/1 -> Sum1/2  "LceHAM"
  positive half2/1 -> Divide5/1  "del_lce"
  Constant5/1 -> Sum10/1
  Divide22/1 -> Sum10/2
  a_tgt/1 -> Sum2/1
  Demux1/1 -> Sum2/2  "a_del"
  Sum2/1 -> Sum3/1  "a_thr"
  Demux1/2 -> Sum3/2  "aRef_HAM"
  Sum3/1 -> Divide22/1
  Demux1/3 -> Divide22/2  "a2lopt_HAM"
  Sum10/1 -> Sum1/1  "lceOffHAM"
  Demux1/4 -> Divide5/2  "LGainHAM"
  Divide5/1 -> Sum4/1, SHAM_Sw_kiii/1  "S_HAM"
  Sum4/1 -> positive half1/1
  Demux1/5 -> Sum4/2  "SHAM_thr"
  positive half1/1 -> Divide1/1, Divide2/1
  Demux1/6 -> Divide1/2  "SGainHAM_KFL"
  Divide1/1 -> SKFL_Sw_kiii/1
  Divide2/1 -> SGAS_Sw_kiii/1
  Demux1/7 -> Divide2/2  "SGainHAM_GAS"

== system nms_sim_2D_cost/Reflex Controller/Lower Control Layer (Spinal Cord)/R Swing Phase/kneeii_damp and hold & kneeiii_leg stop & kneeiv_stance preparation/kneeiv_stance preparation ==
  note: Knee Phase iii
  CtrlPar : Inport
  a_tgt : Inport  Port=2
  LceHFL : Inport  Port=3
  lceGLU : Inport  Port=4
  lceVAS : Inport  Port=5
  Enable : EnablePort  StatesWhenEnabling=reset  ZeroCross=off
  Constant1 : Constant
  Constant2 : Constant
  Constant5 : Constant  Value=pi/2
  Demux2 : Demux  Outputs=8
  Divide{1..3,5..6} (5 alike) : Product
  Sum1 : Sum  Inputs=-+|  InputSameDT=on  SaturateOnIntegerOverflow=on  OutDataTypeStr=Inherit: Same as first input
  Sum2 : Sum  Inputs=++|  InputSameDT=on  SaturateOnIntegerOverflow=on  OutDataTypeStr=Inherit: Same as first input
  Sum3 : Sum  Inputs=+-|  InputSameDT=on  SaturateOnIntegerOverflow=on  OutDataTypeStr=Inherit: Same as first input
  Sum4 : Sum  Inputs=+-|  InputSameDT=on  SaturateOnIntegerOverflow=on  OutDataTypeStr=Inherit: Same as first input
  Sum5 : Sum  Inputs=++|  InputSameDT=on  SaturateOnIntegerOverflow=on  OutDataTypeStr=Inherit: Same as first input
  Sum6 : Sum  Inputs=-+|  InputSameDT=on  SaturateOnIntegerOverflow=on  OutDataTypeStr=Inherit: Same as first input
  Sum7 : Sum  Inputs=+-|  InputSameDT=on  SaturateOnIntegerOverflow=on  OutDataTypeStr=Inherit: Same as first input
  Sum9 : Sum  Inputs=-+|  InputSameDT=on  SaturateOnIntegerOverflow=on  OutDataTypeStr=Inherit: Same as first input
  positive half1 : Saturate  UpperLimit=inf  LowerLimit=0  ZeroCross=off
  positive half2 : Saturate  UpperLimit=inf  LowerLimit=0  ZeroCross=off
  positive half3 : Saturate  UpperLimit=inf  LowerLimit=0  ZeroCross=off
  SHFL_Sw_kiv : Outport  OutputWhenDisabled=reset  InitialOutput=0  VectorParamsAs1DForOutWhenUnconnected=off
  SGLU_Sw_kiv : Outport  Port=2  OutputWhenDisabled=reset  InitialOutput=0  VectorParamsAs1DForOutWhenUnconnected=off
  SVAS_Sw_kiv : Outport  Port=3  OutputWhenDisabled=reset  InitialOutput=0  VectorParamsAs1DForOutWhenUnconnected=off
  wires:
  CtrlPar/1 -> Demux2/1
  Sum1/1 -> positive half2/1
  LceHFL/1 -> Sum1/2
  positive half2/1 -> Divide5/1
  a_tgt/1 -> Sum2/2
  Constant5/1 -> Sum2/1
  Demux2/1 -> Sum3/2  "phiRef_HFL"
  Sum2/1 -> Sum3/1, Sum4/1
  Sum3/1 -> Divide1/1
  Demux2/2 -> Divide1/2  "phi2lopt_HFL"
  Demux2/5 -> Divide2/2  "phi2lopt_GLU"
  Demux2/4 -> Sum4/2  "phiRef_GLU"
  Sum4/1 -> Divide2/1
  Demux2/3 -> Divide5/2  "LGainHFL"
  Divide5/1 -> SHFL_Sw_kiv/1
  Constant1/1 -> Sum5/1
  Divide1/1 -> Sum5/2
  Sum5/1 -> Sum1/1  "lceOffHFL"
  Sum6/1 -> positive half1/1  "del_lce"
  lceGLU/1 -> Sum6/2  "lceGLU"
  positive half1/1 -> Divide3/1
  Demux2/6 -> Divide3/2  "LGainGLU"
  Divide3/1 -> SGLU_Sw_kiv/1
  Constant2/1 -> Sum7/1
  Divide2/1 -> Sum7/2
  Sum7/1 -> Sum6/1  "lceOffGLU"
  Sum9/1 -> positive half3/1
  lceVAS/1 -> Sum9/2
  positive half3/1 -> Divide6/1
  Divide6/1 -> SVAS_Sw_kiv/1
  Demux2/7 -> Sum9/1  "loffVAS"
  Demux2/8 -> Divide6/2  "LGainVAS"
